simulink model "hardware_model_3"  (R2025b)
settings: Solver=FixedStepAuto  StartTime=0.0  StopTime=Inf  FixedStep=t_s  RelTol=1e-3  EnableMultiTasking=on
values from neighbouring files (symbols this model uses):
  c2t = 1 / (k_enc * r_enc)    (= -5.58623066539e-06)    [hardware_init.m]    (also in static_init.m)
  t_s = .0005    (= 0.0005)    [hardware_init.m]    (also in static_init.m)
  V_max = 6.4512    [hardware_init.m]    (also in static_init.m)
undefined symbols (not defined in the file or in its folder): DiscIntNeverNeededParam, Down, GPTRIP1SEL, GPTRIP2SEL, TZ1, TZ2, Up
libraries: c2802xlib x2, c280xlib x1
settings Model: ExtModeTrigDuration=8  Creator=KnaZ  LastModifiedBy=KnaZ
settings OptimizationCC: DefaultUnderspecifiedDataType=single  EnhancedBackFolding=on  PassReuseOutputArgsAs=Individual arguments  MaxStackSize=1024  OptimizeBlockOrder=speed  DifferentSizesBufferReuse=on  OptimizationCustomize=off  EfficientTunableParamExpr=on
settings DebuggingCC: ParameterTunabilityLossMsg=error
settings HardwareCC: ProdBitPerChar=16.0  ProdBitPerInt=16.0  ProdBitPerPointer=32.0  ProdBitPerSizeT=32.0  ProdBitPerPtrDiffT=32.0  ProdLargestAtomicInteger=Integer  ProdLargestAtomicFloat=None  ProdWordSize=16.0  ProdLongLongMode=on  ProdHWDeviceType=Texas Instruments->C2000  HardwareBoardFeatureSet=SoCBlockset
settings SFSimCC: MATLABDynamicMemAlloc=off
settings RTWCC: SystemTargetFile=ert.tlc  HardwareBoard=TI Delfino F28379D LaunchPad  TemplateMakefile=ert_default_tmf  Toolchain=Texas Instruments Code Composer Studio (C2000)  CodeProfilingSaveOptions=MetricsOnly  Description=Embedded Coder
settings CodeAppCC: ForceParamTrailComments=on  IgnoreCustomStorageClasses=off  OperatorAnnotations=on  SimulinkDataObjDesc=on  SFDataObjDesc=on  InsertBlockDesc=on
settings ERTTargetCC: ExtModeTransport=4.0  ExtModeStaticAlloc=on  ExtModeAutomaticAllocSize=off  ExtModeStaticAllocSize=10000.0  ExtModeMexFile=ext_xcp  ExtModeIntrfLevel=Level2 - Open  InlinedParameterPlacement=Hierarchical  CodeReplacementLibrary=TI C28x

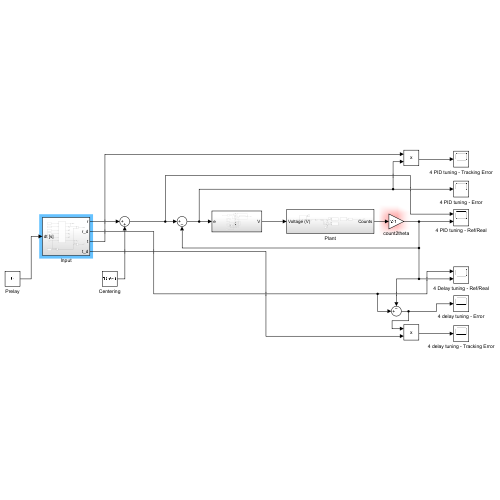
[thumbnail: Simulink's stored preview of the top-level diagram]
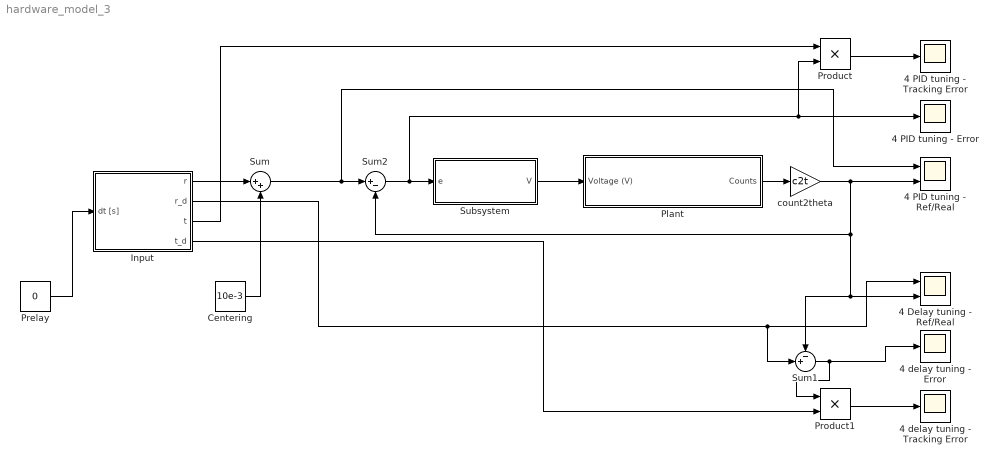
== system hardware_model_3 ==
  4 Delay tuning - Ref/Real : Scope  NumInputPorts=2
      settings: DataLoggingVariableName=ScopeData3
  4 PID tuning - Error : Scope
      settings: ActiveDisplayYMinimum=-0.018629557453095913  ActiveDisplayYMaximum=0.025228350423276424  DataLoggingVariableName=ScopeData2
  4 PID tuning - Ref/Real : Scope  NumInputPorts=2
      settings: ActiveDisplayYMinimum=-0.011874048737809062  ActiveDisplayYMaximum=0.031874892069026828
  4 PID tuning - Tracking Error : Scope
      settings: ActiveDisplayYMinimum=-0.018629557453095913  ActiveDisplayYMaximum=0.025228350423276424  DataLoggingVariableName=ScopeData5
  4 delay tuning - Error : Scope
      settings: ActiveDisplayYMinimum=-0.018629557453095913  ActiveDisplayYMaximum=0.025228350423276424  DataLoggingVariableName=ScopeData4
  4 delay tuning - Tracking Error : Scope
      settings: ActiveDisplayYMinimum=-0.018629557453095913  ActiveDisplayYMaximum=0.025228350423276424  DataLoggingVariableName=ScopeData6
  Centering : Constant  Value=10e-3
  Input : Subsystem
  "Plant " : Subsystem
  Prelay : Constant  Value=0
  Product : Product
  Product1 : Product
  Subsystem : Subsystem
  Sum : Sum  Inputs=|++
  Sum1 : Sum  Inputs=-+|
  Sum2 : Sum  Inputs=|+-
  count2theta : Gain  Gain=c2t
  wires:
  Sum/1 -> 4 PID tuning - Ref/Real/1, Sum2/1
  count2theta/1 -> 4 PID tuning - Ref/Real/2, Sum1/1, 4 Delay tuning - Ref/Real/2, Sum2/2
  Sum2/1 -> Subsystem/1(e), Product/2, 4 PID tuning - Error/1
  "Plant "/1(Counts) -> count2theta/1
  Subsystem/1(V) -> "Plant "/1("Voltage (V) ")
  Input/1(r) -> Sum/1
  Centering/1 -> Sum/2
  Prelay/1 -> Input/1(dt [s])
  Input/2(r_d) -> Sum1/2, 4 Delay tuning - Ref/Real/1
  Sum1/1 -> Product1/1, 4 delay tuning - Error/1
  Product/1 -> 4 PID tuning - Tracking Error/1
  Input/3(t) -> Product/1
  Product1/1 -> 4 delay tuning - Tracking Error/1
  Input/4(t_d) -> Product1/2

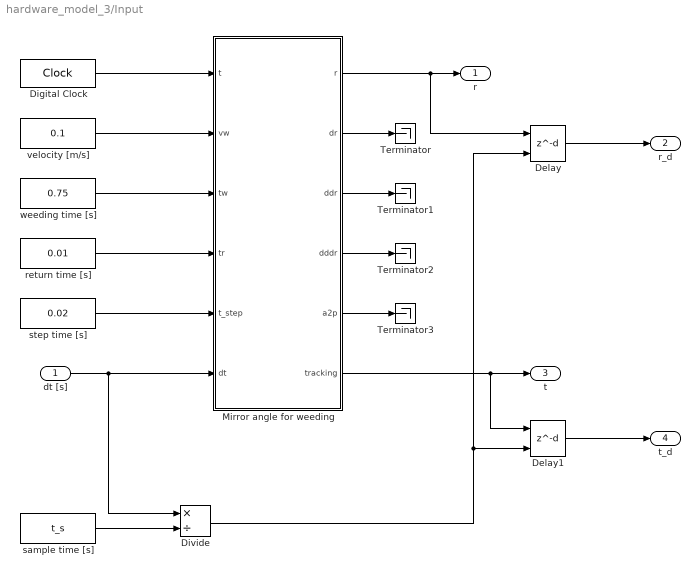
== system hardware_model_3/Input ==
  dt [s] : Inport
  Delay : Delay  DelayLengthSource=Input port  SampleTime=t_s
      settings: InputPortMap=u0,p1
  Delay1 : Delay  DelayLengthSource=Input port  SampleTime=t_s
      settings: InputPortMap=u0,p1
  Digital Clock : DigitalClock  SampleTime=t_s
  Divide : Product  Inputs=*/
  Mirror angle for weeding : MATLAB Function  TreatAsAtomicUnit=on
  Terminator{,1..3} (4 alike) : Terminator
  return time [s] : Constant  Value=0.01  SampleTime=t_s
  sample time [s] : Constant  Value=t_s  SampleTime=t_s
  step time [s] : Constant  Value=0.02
  velocity [m/s] : Constant  Value=0.1  SampleTime=t_s
  weeding time [s] : Constant  Value=0.75  SampleTime=t_s
  r : Outport
  r_d : Outport  Port=2
  t : Outport  Port=3
  t_d : Outport  Port=4
  wires:
  Digital Clock/1 -> Mirror angle for weeding/1(t)
  step time [s]/1 -> Mirror angle for weeding/5(t_step)
  dt [s]/1 -> Divide/1, Mirror angle for weeding/6(dt)
  weeding time [s]/1 -> Mirror angle for weeding/3(tw)
  return time [s]/1 -> Mirror angle for weeding/4(tr)
  sample time [s]/1 -> Divide/2
  Mirror angle for weeding/3(ddr) -> Terminator1/1
  Mirror angle for weeding/5(a2p) -> Terminator3/1
  Mirror angle for weeding/4(dddr) -> Terminator2/1
  velocity [m/s]/1 -> Mirror angle for weeding/2(vw)
  Mirror angle for weeding/2(dr) -> Terminator/1
  Mirror angle for weeding/1(r) -> Delay/1, r/1
  Delay/1 -> r_d/1
  Divide/1 -> Delay1/2, Delay/2
  Mirror angle for weeding/6(tracking) -> Delay1/1, t/1
  Delay1/1 -> t_d/1

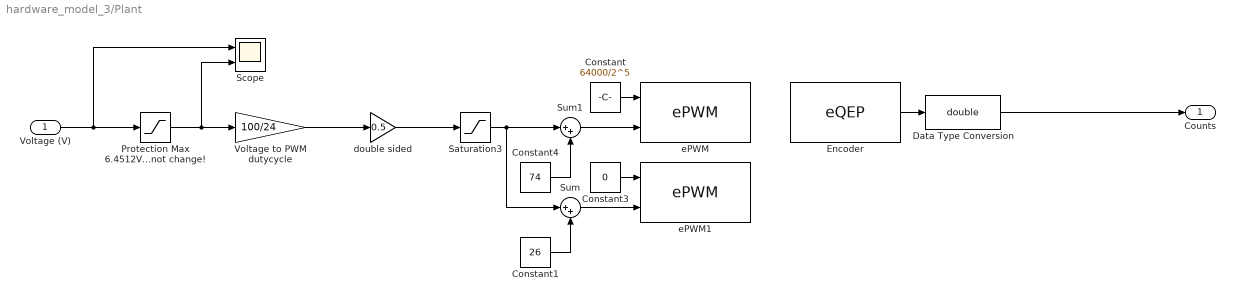
== system hardware_model_3/Plant  ==
  "Voltage (V) " : Inport
  Constant : Constant  Value=64000/2^5
  Constant1 : Constant  Value=26
  Constant3 : Constant  Value=0
  Constant4 : Constant  Value=74
  Data Type Conversion : DataTypeConversion  OutDataTypeStr=double  SaturateOnIntegerOverflow=off  RndMeth=Floor
  Encoder : c280xlib/eQEP  useModule=eQEP2  pcInputmode=Quadrature-count  externalClockrate=2x resolution: Count the rising/falling edge  swapPolarityselection=Clockwise  qdfOutputport=off  qapPolarityselection=off  qbpPolarityselection=off  qipPolarityselection=off  qspPolarityselection=off  igatePolarityselection=off  sampleTime=0.0005  pcOutputport=on  pcMaximumvalue=4294967295  indexInitializationcheck=off  indexInitializationevent=Rising edge  strobeInitializationcheck=off  strobeInitializationevent=Rising edge  softwareInitializationcheck=off  softwareInitializationsource=Set to init value at start up  softwareInitializationmode=on  pcInitialvalue=2147483648  pcResetmode=Reset on the maximum position  ieloutputport=off  indexEventlatch=Rising edge  seloutputport=off  strobeEventlatch=Rising edge  pcefOutputport=off  enableEqepcapture=off  qctmrOutputport=off  qcprdOutputport=off  captureTimerprescaler=128  upEventprescaler=128  overflowErrorflag=off  directionErrorflag=off  captureTimerposition=On position counter read  unitTimerperiod=100000000  captureTimerlatch=off  capturePeriodlatch=off  positionCounterlatch=off  soenPolarityselection=off  spselPolarityselection=Index pin is used for sync output  compareValuesource=Specify via dialog  shadowMode=Load on QPOSCNT=0  compareValue=4294967295  syncOutputwidth=1  polaritySyncoutput=Active high  watchdogEnable=off  watchdogTimer=65535  outport1Datatype=auto  outport2Datatype=int32  outport3Datatype=auto  outport4Datatype=auto  outport5Datatype=auto  outport6Datatype=auto  outport7Datatype=auto  outport8Datatype=auto  outport9Datatype=auto  outport10Datatype=auto  outport11Datatype=auto  outport12Datatype=auto  eqepinterrupt_pce=off  eqepinterrupt_qpe=off  eqepinterrupt_qdc=off  eqepinterrupt_wto=off  eqepinterrupt_pcu=off  eqepinterrupt_pco=off  eqepinterrupt_pcr=off  eqepinterrupt_pcm=off  eqepinterrupt_sel=off  eqepinterrupt_iel=off  eqepinterrupt_uto=off  pheOutputport=off  watchdogOutputport=off  outport13Datatype=auto  outport14Datatype=auto
  Protection Max 6.4512V Do not change! : Saturate  UpperLimit=6.4512  LowerLimit=-6.4512
  Saturation3 : Saturate  UpperLimit=25  LowerLimit=-25
  Scope : Scope  NumInputPorts=2
      settings: ActiveDisplayYMinimum=5.30194765329361  ActiveDisplayYMaximum=5.4454273581504822
  Sum : Sum  Inputs=|++
  Sum1 : Sum  Inputs=|++
  Voltage to PWM dutycycle : Gain  Gain=100/24
  double sided : Gain  Gain=0.5
  ePWM : c2802xlib/ePWM  PwmType=C2000_Type4  useModule=ePWM4  ePWMxLINKTBPRD=Not Linked  periodUnits=Clock cycles  timerSource=Input port  timerPeriod_clk=64000  timerPeriod_sec=0.0000050  tbshadow=Counter equals to zero  countingMode=Up-Down  phaseActiveEnable=Disable  phaseDirection=Count down after sync  phaseActive=0  synchronizationEnable=off  dcaevt1Sync=off  dcbevt1Sync=off  synchronizationOption=Counter equals to zero (CTR=Zero)  dcbevt1SyncOut=off  dcaevt1SyncOut=off  cmpdSyncOut=off  cmpcSyncOut=off  cmpbSyncOut=off  zeroSyncOut=on  swfSyncOut=off  perSynchronizationOption=Counter equals to period (CTR=PRD)  clockPrescale=1  HSclockPrescale=1  enswap=off  ePWMxAStatus=on  ePWMxAactionLogic1=Set  ePWMxAactionLogic2=Clear  ePWMxAactionLogic3=Clear  ePWMxAactionLogic4=Set  ePWMxAactionLogic5=Do nothing  ePWMxAactionLogic6=Do nothing  ePWMxACSFenable=off  ePWMxACSFvalue=Forcing disable  ePWMxASFreload=Zero  ePWMxBStatus=off  ePWMxBactionLogic1=Set  ePWMxBactionLogic2=Clear  ePWMxBactionLogic3=Do nothing  ePWMxBactionLogic4=Do nothing  ePWMxBactionLogic5=Clear  ePWMxBactionLogic6=Set  ePWMxBCSFenable=off  ePWMxBCSFvalue=Forcing disable  ePWMxBSFreload=Zero  ePWNxBOutWay=off  ePWMxLINKCMPA=Not Linked  CMPAUnits=Percentages  CMPASource=Input port  CMPAValue_per=50  CMPAValue_clk=32000  enCMPAshadow=Counter equals to zero (CTR=Zero)  ePWMxLINKCMPB=Not Linked  CMPBUnits=Clock cycles  CMPBSource=Specify via dialog  CMPBValue_per=50  CMPBValue_clk=32000  enCMPBshadow=Counter equals to zero (CTR=Zero)  ePWMxLINKCMPC=Not Linked  CMPCUnits=Clock cycles  CMPCSource=Specify via dialog  CMPCValue_per=50  CMPCValue_clk=32000  enCMPCshadow=Counter equals to zero (CTR=Zero)  ePWMxLINKCMPD=Not Linked  CMPDUnits=Clock cycles  CMPDSource=Specify via dialog  CMPDValue_per=50  CMPDValue_clk=32000  enCMPDshadow=Counter equals to zero (CTR=Zero)  enableDBePWMxA=off  enableDBePWMxB=off  enhalfcycle=off  DBpolarity=Active high (AH)  DBedgeDelay=Positive  DBSource_ePWMxA=ePWMxA  DBSource_ePWMxB=ePWMxA  DBPeriodUnits=Clock cycles  DBperiodSource=Specify via dialog  REDperiod=0  FEDperiod=0  REDperiod_sec=0  FEDperiod_sec=0  LoadModeDBRED=Immediate without using shadow  LoadModeDBFED=Immediate without using shadow  adcstartModuleA=off  adcrequestEventA=First event  adcstartEventA=Digital Compare Module A Event 1 start of conversion (DCAEVT1.soc)  adcstartEventA_type2=Digital Compare Module A Event 1 start of conversion (DCAEVT1.soc)  adcstartModuleB=off  adcrequestEventB=First event  adcstartEventB=Counter equals to zero (CTR=Zero)  adcstartEventB_type2=Counter equals to zero (CTR=Zero)  intEn=off  intPrd=First event  intSel=Counter equals to zero (CTR=Zero)  intSel_type2=Counter equals to zero (CTR=Zero)  hrpe=off  enHRPWM=off  HRPWM_LoadMode=Counter equals to period (CTR=PRD)  HRPWM_CTLMode=Duty or Period control mode  HRPWM_EDGMode=Both edge  hrpeb=off  enHRPWMB=off  HRPWM_LoadModeB=Counter equals to zero (CTR=ZERO)  HRPWM_CTLModeB=Duty or Period control mode  HRPWM_EDGModeB=Both edge  enHRDBRED=off  enHRDBFED=off  enSFO=on  enautoconv=on  chopperEnable=off  chopperFrequency=1  chopperFirstwidth=1  chopperDuty=12.5%  tripZonesource=Specify via dialog  tzselOSHT1=off  tzselOSHT2=off  tzselOSHT3=off  tzselOSHT4=off  tzselOSHT5=off  tzselOSHT6=off  tzselOSHDCAEV1=off  tzselOSHDCBEV1=off  tzselCBC1=off  tzselCBC2=off  tzselCBC3=off  tzselCBC4=off  tzselCBC5=off  tzselCBC6=off  tzselCBCDCAEV2=off  tzselCBCDCBEV2=off  enTzOstIntr=off  enTzCbcIntr=off  enTzDCAEVT1Intr=off  enTzDCAEVT2Intr=off  enTzDCBEVT1Intr=off  enTzDCBEVT2Intr=off  tzclrCBCLatch=Counter equals to zero (CTR=Zero)  ePWMxAforced=No action  ePWMxBforced=No action  DCAEVT1forced=No action  DCBEVT1forced=No action  DCAEVT2forced=No action  DCBEVT2forced=No action  dcah=Trip Zone 1 input (TZ1)  dcal=Trip Zone 2 input (TZ2)  dcbh=Trip Zone 1 input (TZ1)  dcbl=Trip Zone 2 input (TZ2)  dcah_type2=GPTRIP1SEL/(TZ1)  dcal_type2=GPTRIP2SEL/(TZ2)  dcbh_type2=GPTRIP1SEL/(TZ1)  dcbl_type2=GPTRIP2SEL/(TZ2)  gendcaevt1=Event disabled  gendcaevt2=Event disabled  gendcbevt1=Event disabled  gendcbevt2=Event disabled  dcaevt1src=DCAEVT1 with sync  dcaevt2src=DCAEVT2 with sync  dcbevt1src=DCBEVT1 with sync  dcbevt2src=DCBEVT2 with sync  pulsesel=Counter equals to zero (CTR=Zero)  blankinv=off  blankoffset=0  blankwidth=0  evsrcsel=Filtered version of DCAEVT1 (DCAEVT1FILT)  encape=off
  ePWM1 : c2802xlib/ePWM  PwmType=C2000_Type4  useModule=ePWM5  ePWMxLINKTBPRD=ePWM4  periodUnits=Clock cycles  timerSource=Specify via dialog  timerPeriod_clk=64000  timerPeriod_sec=0.0000025  tbshadow=Counter equals to zero  countingMode=Up-Down  phaseActiveEnable=Set counter to phase value specified via input port  phaseDirection=Count up after sync  phaseActive=0  synchronizationEnable=off  dcaevt1Sync=off  dcbevt1Sync=off  synchronizationOption=Pass through (EPWMxSYNCI or SWFSYNC)  dcbevt1SyncOut=off  dcaevt1SyncOut=off  cmpdSyncOut=off  cmpcSyncOut=off  cmpbSyncOut=off  zeroSyncOut=off  swfSyncOut=on  perSynchronizationOption=Counter equals to period (CTR=PRD)  clockPrescale=1  HSclockPrescale=1  enswap=off  ePWMxAStatus=on  ePWMxAactionLogic1=Clear  ePWMxAactionLogic2=Set  ePWMxAactionLogic3=Set  ePWMxAactionLogic4=Clear  ePWMxAactionLogic5=Do nothing  ePWMxAactionLogic6=Do nothing  ePWMxACSFenable=off  ePWMxACSFvalue=Forcing disable  ePWMxASFreload=Zero  ePWMxBStatus=off  ePWMxBactionLogic1=Set  ePWMxBactionLogic2=Clear  ePWMxBactionLogic3=Do nothing  ePWMxBactionLogic4=Do nothing  ePWMxBactionLogic5=Clear  ePWMxBactionLogic6=Set  ePWMxBCSFenable=off  ePWMxBCSFvalue=Forcing disable  ePWMxBSFreload=Zero  ePWNxBOutWay=off  ePWMxLINKCMPA=Not Linked  CMPAUnits=Percentages  CMPASource=Input port  CMPAValue_per=50  CMPAValue_clk=32000  enCMPAshadow=Counter equals to zero (CTR=Zero)  ePWMxLINKCMPB=Not Linked  CMPBUnits=Clock cycles  CMPBSource=Specify via dialog  CMPBValue_per=50  CMPBValue_clk=32000  enCMPBshadow=Counter equals to zero (CTR=Zero)  ePWMxLINKCMPC=Not Linked  CMPCUnits=Clock cycles  CMPCSource=Specify via dialog  CMPCValue_per=50  CMPCValue_clk=32000  enCMPCshadow=Counter equals to zero (CTR=Zero)  ePWMxLINKCMPD=Not Linked  CMPDUnits=Clock cycles  CMPDSource=Specify via dialog  CMPDValue_per=50  CMPDValue_clk=32000  enCMPDshadow=Counter equals to zero (CTR=Zero)  enableDBePWMxA=off  enableDBePWMxB=off  enhalfcycle=off  DBpolarity=Active high (AH)  DBedgeDelay=Positive  DBSource_ePWMxA=ePWMxA  DBSource_ePWMxB=ePWMxA  DBPeriodUnits=Clock cycles  DBperiodSource=Specify via dialog  REDperiod=0  FEDperiod=0  REDperiod_sec=0  FEDperiod_sec=0  LoadModeDBRED=Immediate without using shadow  LoadModeDBFED=Immediate without using shadow  adcstartModuleA=off  adcrequestEventA=First event  adcstartEventA=Digital Compare Module A Event 1 start of conversion (DCAEVT1.soc)  adcstartEventA_type2=Digital Compare Module A Event 1 start of conversion (DCAEVT1.soc)  adcstartModuleB=off  adcrequestEventB=First event  adcstartEventB=Counter equals to zero (CTR=Zero)  adcstartEventB_type2=Counter equals to zero (CTR=Zero)  intEn=off  intPrd=First event  intSel=Counter equals to zero (CTR=Zero)  intSel_type2=Counter equals to zero (CTR=Zero)  hrpe=off  enHRPWM=off  HRPWM_LoadMode=Counter equals to period (CTR=PRD)  HRPWM_CTLMode=Duty or Period control mode  HRPWM_EDGMode=Both edge  hrpeb=off  enHRPWMB=off  HRPWM_LoadModeB=Counter equals to zero (CTR=ZERO)  HRPWM_CTLModeB=Duty or Period control mode  HRPWM_EDGModeB=Both edge  enHRDBRED=off  enHRDBFED=off  enSFO=on  enautoconv=on  chopperEnable=off  chopperFrequency=1  chopperFirstwidth=1  chopperDuty=12.5%  tripZonesource=Specify via dialog  tzselOSHT1=off  tzselOSHT2=off  tzselOSHT3=off  tzselOSHT4=off  tzselOSHT5=off  tzselOSHT6=off  tzselOSHDCAEV1=off  tzselOSHDCBEV1=off  tzselCBC1=off  tzselCBC2=off  tzselCBC3=off  tzselCBC4=off  tzselCBC5=off  tzselCBC6=off  tzselCBCDCAEV2=off  tzselCBCDCBEV2=off  enTzOstIntr=off  enTzCbcIntr=off  enTzDCAEVT1Intr=off  enTzDCAEVT2Intr=off  enTzDCBEVT1Intr=off  enTzDCBEVT2Intr=off  tzclrCBCLatch=Counter equals to zero (CTR=Zero)  ePWMxAforced=No action  ePWMxBforced=No action  DCAEVT1forced=No action  DCBEVT1forced=No action  DCAEVT2forced=No action  DCBEVT2forced=No action  dcah=Trip Zone 1 input (TZ1)  dcal=Trip Zone 2 input (TZ2)  dcbh=Trip Zone 1 input (TZ1)  dcbl=Trip Zone 2 input (TZ2)  dcah_type2=GPTRIP1SEL/(TZ1)  dcal_type2=GPTRIP2SEL/(TZ2)  dcbh_type2=GPTRIP1SEL/(TZ1)  dcbl_type2=GPTRIP2SEL/(TZ2)  gendcaevt1=Event disabled  gendcaevt2=Event disabled  gendcbevt1=Event disabled  gendcbevt2=Event disabled  dcaevt1src=DCAEVT1 with sync  dcaevt2src=DCAEVT2 with sync  dcbevt1src=DCBEVT1 with sync  dcbevt2src=DCBEVT2 with sync  pulsesel=Counter equals to zero (CTR=Zero)  blankinv=off  blankoffset=0  blankwidth=0  evsrcsel=Filtered version of DCAEVT1 (DCAEVT1FILT)  encape=off
  Counts : Outport  VectorParamsAs1DForOutWhenUnconnected=off
  wires:
  Data Type Conversion/1 -> Counts/1
  Encoder/1 -> Data Type Conversion/1
  "Voltage (V) "/1 -> Scope/1, Protection Max 6.4512V Do not change!/1
  Constant1/1 -> Sum/2
  Constant3/1 -> ePWM1/1
  Sum/1 -> ePWM1/2
  Protection Max 6.4512V Do not change!/1 -> Scope/2, Voltage to PWM dutycycle/1
  Constant/1 -> ePWM/1
  Constant4/1 -> Sum1/2
  Saturation3/1 -> Sum/1, Sum1/1
  Sum1/1 -> ePWM/2
  Voltage to PWM dutycycle/1 -> double sided/1
  double sided/1 -> Saturation3/1

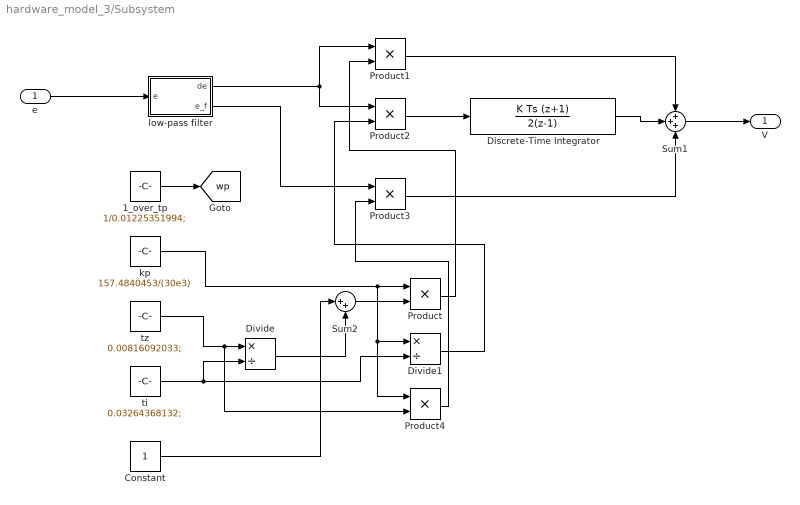
== system hardware_model_3/Subsystem ==
  e : Inport
  1_over_tp : Constant  Value=1/0.01225351994;  SampleTime=t_s
  Constant : Constant
  Discrete-Time Integrator : DiscreteIntegrator  IntegratorMethod=Integration: Trapezoidal  SampleTime=t_s  LimitOutput=on  UpperSaturationLimit=V_max  LowerSaturationLimit=-V_max  ICPrevOutput=DiscIntNeverNeededParam  ICPrevScaledInput=DiscIntNeverNeededParam
  Divide : Product  Inputs=*/
  Divide1 : Product  Inputs=*/
  Product{,1..4} (5 alike) : Product
  Sum1 : Sum  Inputs=+++
  Sum2 : Sum  Inputs=|++
  kp : Constant  Value=157.4840453/(30e3)
  low-pass filter : Subsystem
  ti : Constant  Value=0.03264368132;
  tz : Constant  Value=0.00816092033;
  V : Outport
  tag scope: wp=global
  wires:
  Product2/1 -> Discrete-Time Integrator/1
  low-pass filter/2(e_f) -> Product3/1
  Discrete-Time Integrator/1 -> Sum1/2
  Product1/1 -> Sum1/1
  1_over_tp/1 -> [wp]
  Product3/1 -> Sum1/3
  low-pass filter/1(de) -> Product2/1, Product1/1
  Sum1/1 -> V/1
  e/1 -> low-pass filter/1(e)
  Constant/1 -> Sum2/1
  Sum2/1 -> Product/2
  kp/1 -> Divide1/1, Product4/1, Product/1
  tz/1 -> Product4/2, Divide/1
  ti/1 -> Divide1/2, Divide/2
  Divide/1 -> Sum2/2
  Product/1 -> Product1/2
  Divide1/1 -> Product2/2
  Product4/1 -> Product3/2

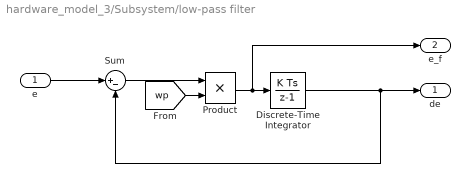
== system hardware_model_3/Subsystem/low-pass filter ==
  e : Inport
  Discrete-Time Integrator : DiscreteIntegrator  SampleTime=t_s  ICPrevOutput=DiscIntNeverNeededParam  ICPrevScaledInput=DiscIntNeverNeededParam
  Product : Product
  Sum : Sum  Inputs=|+-
  de : Outport
  e_f : Outport  Port=2
  wires:
  e/1 -> Sum/1
  Product/1 -> e_f/1, Discrete-Time Integrator/1
  Sum/1 -> Product/1
  [wp] -> Product/2
  Discrete-Time Integrator/1 -> de/1, Sum/2

== matlab function hardware_model_3/Input/Mirror angle for weeding ==
  data: t input; vw input; tw input; tr input; t_step input; r output; dr output; ddr output; dddr output; a2p output; dt input; tracking output
function [r, dr, ddr, dddr, a2p, tracking] = Trajectory(t, vw, tw, tr, t_step, dt)
% Generates the mirror angle trajectory for weeding
% OUTPUTS:
%   r:     [rad]     angle
%   dr:    [rad/s]   angular velocity
%   ddr:   [rad/s^2] angular acceleration
%   dddr:  [rad/s^3] angular jerk
%   a2p:   [m/rad]   angle to position transmission
% INPUTS
%   t:      [s] master clock (from Simulink Clock block)
%   vw:     [m/s] driving velocity
%   tw:     [s] weeding time
%   tr:     [s] return time
%   ts:     [s] sample time (unused now, kept for interface)
%   t_step: [s] dwell time at min value between return and weeding
%   dt:     [s] preplay lead time

% ---- preplay: evaluate trajectory ahead by dt ----
Tp = tw + tr + t_step;                 % [s] total period
t  = mod(t + dt, Tp);                   % [s] shifted, wrapped time

at = 2*pi/tr;                           % [1/s] angular rate in sine period

% auxiliary variables
D  = vw*(tw+tr);                        % [m] maximum spot amplitude
xs = (D*tw)/(2*(tr + tw)) ...
   + (D*(1 - tw^2/(tr + tw)^2)^(1/2))/(2*pi) ...
   - (D*tw*acos(tw/(tr + tw)))/(2*pi*(tr + tw));  % [m] maximum amplitude
a2p = xs/17.5e-3;                       % [m/rad] angle to position transmission
Da  = D/a2p;                            % [rad] angular amplitude
va  = vw/a2p;                           % [rad/s] angular velocity
a   = Da*tw/(tw+tr)/2;                  % polynomial offset coefficient
b   = -2*a/tr;                          % polynomial slope coefficient
c   = Da/(2*pi);                        % sinusoidal amplitude

% min value the return part ends at (= constant-velocity start value)
r_min = -Da*tw/(tw+tr)/2;

% compute angular trajectory and time derivatives
tracking = 0;
if t <= tr
    % sinusoidal return part
    r    =  a + b*t + c*sin(at*t);
    dr   =  b + c*at*cos(at*t);
    ddr  = -c*at^2*sin(at*t);
    dddr = -c*at^3*cos(at*t);
elseif t <= tr + t_step
    % step: hold at min value
    r    = r_min;
    dr   = 0;
    ddr  = 0;
    dddr = 0;
else
    % constant velocity weeding part
    r    = r_min + (t - tr - t_step)*va;
    dr   = va;
    ddr  = 0;
    dddr = 0;
    tracking = 1;
end
end
